simulink model "fault_ann"  (R2024a)
settings: Solver=VariableStepAuto  StartTime=0.0  StopTime=0.2  RelTol=1e-3
libraries: spsThreePhasePISectionLineLib x2, spsThreePhaseSourceLib x2, spsThreePhaseVIMeasurementLib x1, spsThreePhaseFaultLib x1, sps_lib x1
settings Model: Creator=defaultuser0  LastModifiedBy=defaultuser0

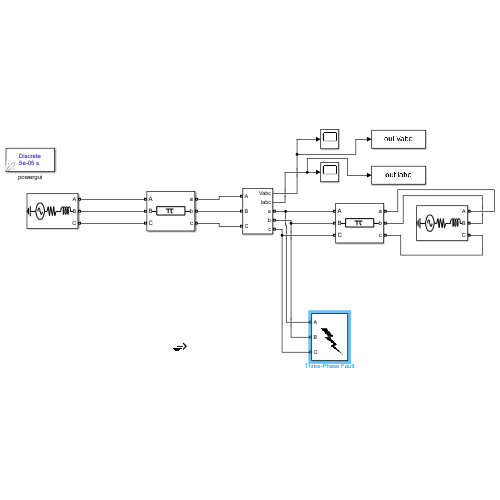
[thumbnail: Simulink's stored preview of the top-level diagram]
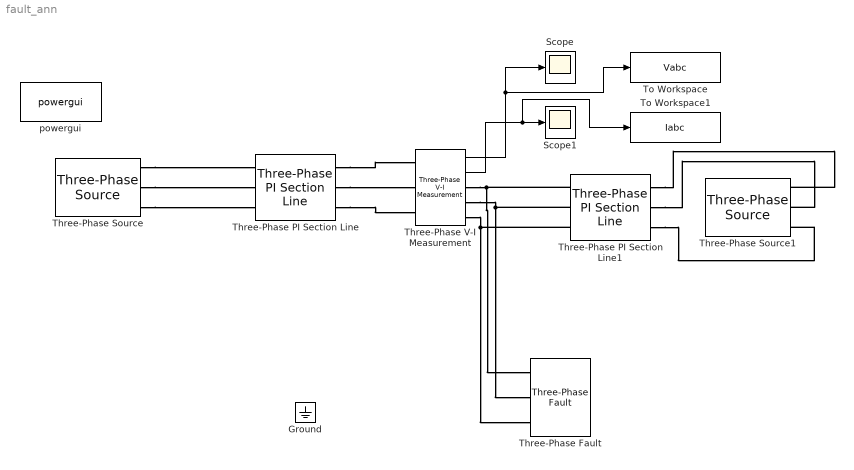
== system fault_ann ==
  Ground : Ground
  Scope : Scope
  Scope1 : Scope
  Three-Phase PI Section Line : spsThreePhasePISectionLineLib/Three-Phase PI Section Line  LConnTagsString=a|b|c  RConnTagsString=A|B|C  Length=100  Frequency=60  Resistances=[ 0.01273 0.3864]  Inductances="[ 0.9337e-3  4.1264e-3]"  Capacitances=[12.74e-9 7.751e-9]
  Three-Phase PI Section Line1 : spsThreePhasePISectionLineLib/Three-Phase PI Section Line  LConnTagsString=a|b|c  RConnTagsString=A|B|C  Length=100  Frequency=50  Resistances=[ 0.01273 0.3864]  Inductances="[ 0.9337e-3  4.1264e-3]"  Capacitances=[12.74e-9 7.751e-9]
  Three-Phase V-I Measurement : spsThreePhaseVIMeasurementLib/Three-Phase V-I Measurement  VoltageMeasurement=phase-to-ground  SetLabelV=off  LabelV=Vabc  Vpu=off  VpuLL=off  CurrentMeasurement=yes  SetLabelI=off  LabelI=Iabc  Ipu=off  Pbase=100e6  Vbase=500e3  OutputType=Complex  PhasorSimulation=off  PSBequivalent=0
  Three-Phase Fault : spsThreePhaseFaultLib/Three-Phase Fault  InitialStates=0  FaultA=on  FaultB=on  FaultC=on  GroundFault=on  SwitchTimes=[0.1 0.15]  External=off  SwitchStatus=NaN  FaultResistance=0.001  GroundResistance=1  SnubberResistance=1e6  SnubberCapacitance=inf  Measurements=Fault voltages and currents
  Three-Phase Source : spsThreePhaseSourceLib/Three-Phase Source  InternalConnection=Yg  VoltagePhases=off  Voltage=11000  PhaseAngle=0  Voltage_phases=[25e3 25e3 25e3]/sqrt(3)  PhaseAngles_phases=[0 -120 +120]  Frequency=50  NonIdealSource=on  SpecifyImpedance=off  Resistance=0.8929  Inductance=16.58e-3  ShortCircuitLevel=100e6  BaseVoltage=11000  XRratio=7  BusType=swing  Pref=10e3  Qref=0  Prefabc=[10e3, 10e3, 10e3]  Qrefabc=[0, 0, 0]  Qmin=-inf  Qmax=inf
  Three-Phase Source1 : spsThreePhaseSourceLib/Three-Phase Source  InternalConnection=Yg  VoltagePhases=off  Voltage=25e3  PhaseAngle=0  Voltage_phases=[25e3 25e3 25e3]/sqrt(3)  PhaseAngles_phases=[0 -120 +120]  Frequency=60  NonIdealSource=on  SpecifyImpedance=off  Resistance=0.8929  Inductance=16.58e-3  ShortCircuitLevel=100e6  BaseVoltage=25e3  XRratio=7  BusType=swing  Pref=10e3  Qref=0  Prefabc=[10e3, 10e3, 10e3]  Qrefabc=[0, 0, 0]  Qmin=-inf  Qmax=inf
  To Workspace : ToWorkspace  VariableName=Vabc  SaveFormat=Timeseries  SampleTime=-1
  To Workspace1 : ToWorkspace  VariableName=Iabc  SaveFormat=Timeseries  SampleTime=-1
  powergui : sps_lib/powergui  Priority=1  SimulationMode=Discrete  SampleTime=50e-6  frequency=60  Iterations=50  frequencyindice=60  Pbase=100e6  ErrMax=1e-4  UnitsV=kV  UnitsW=MW  buscounter=0  FunctionMessages=off  echomessages=off  EnableUseOfTLC=off  CurrentSourceSwitches=off  DisableSnubberDevices=off  DisableRonSwitches=off  DisableVfSwitches=off  DisplayEquations=off  AutomaticDiscreteSolvers=off  SolverType=Tustin/Backward Euler (TBE)  Interpol=off  ExternalGateDelay=off  methode=off  Ts=100  x0status=blocks  SPID=on  SwTol=0  HookPort=off  NonlinearTolerance=1e-4  nMaxIteration=100  ContinueOnMaxIteration=off  RestoreLinks=warning  ResistiveCurrentMeasurement=off  Frange=[0:2:500]  Ylog=off  Xlog=on  ShowGrid=off  save=off  variable=ZData  structure=0  ZoomFFT=off  StartTime=0.0  cycles=1  DisplayStyle=1  fundamental=60  FreqAxis=off  MaxFrequency=1000  frequencyindicesteady=1  RmsSteady=1  display=off
  wires:
  Three-Phase V-I Measurement/1 -> To Workspace/1, Scope/1
  Three-Phase V-I Measurement/2 -> To Workspace1/1, Scope1/1
  connections:
  Three-Phase Source/RConn1 -- Three-Phase PI Section Line/LConn1
  Three-Phase Source/RConn2 -- Three-Phase PI Section Line/LConn2
  Three-Phase Source/RConn3 -- Three-Phase PI Section Line/LConn3
  Three-Phase PI Section Line/RConn1 -- Three-Phase V-I Measurement/LConn1
  Three-Phase PI Section Line/RConn2 -- Three-Phase V-I Measurement/LConn2
  Three-Phase PI Section Line/RConn3 -- Three-Phase V-I Measurement/LConn3
  Three-Phase V-I Measurement/RConn1 -- Three-Phase PI Section Line1/LConn1 -- Three-Phase Fault/LConn1
  Three-Phase V-I Measurement/RConn2 -- Three-Phase PI Section Line1/LConn2 -- Three-Phase Fault/LConn2
  Three-Phase V-I Measurement/RConn3 -- Three-Phase PI Section Line1/LConn3 -- Three-Phase Fault/LConn3
  Three-Phase PI Section Line1/RConn1 -- Three-Phase Source1/RConn1
  Three-Phase PI Section Line1/RConn2 -- Three-Phase Source1/RConn2
  Three-Phase PI Section Line1/RConn3 -- Three-Phase Source1/RConn3
